simulink model "youBot_Arm_recovery"  (R2024a)
settings: Solver=ode15s  StartTime=0.0  StopTime=20  MaxStep=1e-2  RelTol=1e-3  AbsTol=1e-4
model workspace: external: MATLAB File youBot_DataFile.m (data not in the file)
undefined symbols (not defined in the file): Extr_Data_LinkHoles, Qt, s_curve_home2in, s_curve_in2out, s_curve_out2home, sigbuilder_block, smiData, X, Y, YBT_Par, Z
libraries: sm_lib x193, nesl_utility x130, fl_lib x53, simulink x13, Parts_Lib x10, MyMath_lib x8, Motor_Lib x5, Contact_Forces_Lib x4, ee_lib x2, sdl_lib x2
(part 8 of 8)

== system youBot_Arm_recovery/Arm/Environment/Conveyors/Belt In/Light Curtain/Geometry ==
  Beam 1 : sm_lib/Body Elements/Cylindrical Solid  CylinderRadius=beam_radius  CylinderRadiusUnits=m  CylinderLength=beam_length  CylinderLengthUnits=m  ExportEntireGeometry=off  InertiaType=CalculateFromGeometry  BasedOnType=Density  Density=1  DensityUnits=kg/m^3  Mass=1  MassUnits=kg  CenterOfMass=[0 0 0]  CenterOfMassUnits=m  MomentsOfInertia=[1 1 1]  MomentsOfInertiaUnits=kg*m^2  ProductsOfInertia=[1 1 1]  ProductsOfInertiaUnits=kg*m^2  GraphicType=FromGeometry  MarkerShape=Sphere  MarkerSize=10  GraphicVisPropType=SimpleVisualProperties  GraphicDiffuseColor=beam_color  GraphicOpacity=beam_opc  GraphicSpecularColor=[0.5 0.5 0.5 1.0]  GraphicAmbientColor=[0.15 0.15 0.15 1.0]  GraphicEmissiveColor=[0.0 0.0 0.0 1.0]  GraphicShininess=75  DoExposeReferenceFrame=on  SerializedFrames=<Frames/>
  Beam 2 : sm_lib/Body Elements/Cylindrical Solid  CylinderRadius=beam_radius  CylinderRadiusUnits=m  CylinderLength=beam_length  CylinderLengthUnits=m  ExportEntireGeometry=off  InertiaType=CalculateFromGeometry  BasedOnType=Density  Density=1  DensityUnits=kg/m^3  Mass=1  MassUnits=kg  CenterOfMass=[0 0 0]  CenterOfMassUnits=m  MomentsOfInertia=[1 1 1]  MomentsOfInertiaUnits=kg*m^2  ProductsOfInertia=[1 1 1]  ProductsOfInertiaUnits=kg*m^2  GraphicType=FromGeometry  MarkerShape=Sphere  MarkerSize=10  GraphicVisPropType=SimpleVisualProperties  GraphicDiffuseColor=beam_color  GraphicOpacity=beam_opc  GraphicSpecularColor=[0.5 0.5 0.5 1.0]  GraphicAmbientColor=[0.15 0.15 0.15 1.0]  GraphicEmissiveColor=[0.0 0.0 0.0 1.0]  GraphicShininess=75  DoExposeReferenceFrame=on  SerializedFrames=<Frames/>
  Beam 3 : sm_lib/Body Elements/Cylindrical Solid  CylinderRadius=beam_radius  CylinderRadiusUnits=m  CylinderLength=beam_length  CylinderLengthUnits=m  ExportEntireGeometry=off  InertiaType=CalculateFromGeometry  BasedOnType=Density  Density=1  DensityUnits=kg/m^3  Mass=1  MassUnits=kg  CenterOfMass=[0 0 0]  CenterOfMassUnits=m  MomentsOfInertia=[1 1 1]  MomentsOfInertiaUnits=kg*m^2  ProductsOfInertia=[1 1 1]  ProductsOfInertiaUnits=kg*m^2  GraphicType=FromGeometry  MarkerShape=Sphere  MarkerSize=10  GraphicVisPropType=SimpleVisualProperties  GraphicDiffuseColor=beam_color  GraphicOpacity=beam_opc  GraphicSpecularColor=[0.5 0.5 0.5 1.0]  GraphicAmbientColor=[0.15 0.15 0.15 1.0]  GraphicEmissiveColor=[0.0 0.0 0.0 1.0]  GraphicShininess=75  DoExposeReferenceFrame=on  SerializedFrames=<Frames/>
  Transform Beam 1 : sm_lib/Frames and Transforms/Rigid Transform  RotationMethod=None  FollAlignAxisA=+X  BaseAlignAxisA=+Y  FollAlignAxisB=+Y  BaseAlignAxisB=+Z  RotationStandardAxis=+Z  RotationAngle=0.0  RotationAngleUnits=deg  RotationArbitraryAxis=[0 0 1]  RotationSequenceAxes=FollowerAxes  RotationSequence=XYX  RotationSequenceAngles=[0 0 0]  RotationSequenceAnglesUnits=deg  RotationMatrix=[1 0 0; 0 1 0; 0 0 1]  Quaternion=[1 0 0 0]  TranslationMethod=StandardAxis  TranslationCartesianOffset=[0 0 0]  TranslationCartesianOffsetUnits=m  TranslationStandardAxis=-X  TranslationStandardOffset=YBT_Par.BeltIn.Sensor.Beam.offset  TranslationStandardOffsetUnits=m  TranslationROffset=0  TranslationROffsetUnits=m  TranslationThetaOffset=0  TranslationThetaOffsetUnits=deg  TranslationZOffset=0  TranslationZOffsetUnits=m
  Transform Beam 3 : sm_lib/Frames and Transforms/Rigid Transform  RotationMethod=None  FollAlignAxisA=+X  BaseAlignAxisA=+Y  FollAlignAxisB=+Y  BaseAlignAxisB=+Z  RotationStandardAxis=+Z  RotationAngle=0.0  RotationAngleUnits=deg  RotationArbitraryAxis=[0 0 1]  RotationSequenceAxes=FollowerAxes  RotationSequence=XYX  RotationSequenceAngles=[0 0 0]  RotationSequenceAnglesUnits=deg  RotationMatrix=[1 0 0; 0 1 0; 0 0 1]  Quaternion=[1 0 0 0]  TranslationMethod=StandardAxis  TranslationCartesianOffset=[0 0 0]  TranslationCartesianOffsetUnits=m  TranslationStandardAxis=-X  TranslationStandardOffset=YBT_Par.BeltIn.Sensor.Beam.offset  TranslationStandardOffsetUnits=m  TranslationROffset=0  TranslationROffsetUnits=m  TranslationThetaOffset=0  TranslationThetaOffsetUnits=deg  TranslationZOffset=0  TranslationZOffsetUnits=m
  Transform Orient z : sm_lib/Frames and Transforms/Rigid Transform  RotationMethod=AlignedAxes  FollAlignAxisA=+X  BaseAlignAxisA=+Z  FollAlignAxisB=+Z  BaseAlignAxisB=+Y  RotationStandardAxis=+X  RotationAngle=90  RotationAngleUnits=deg  RotationArbitraryAxis=[0 0 1]  RotationSequenceAxes=FollowerAxes  RotationSequence=XYX  RotationSequenceAngles=[0 0 0]  RotationSequenceAnglesUnits=deg  RotationMatrix=[1 0 0; 0 1 0; 0 0 1]  Quaternion=[1 0 0 0]  TranslationMethod=None  TranslationCartesianOffset=[0 0 0]  TranslationCartesianOffsetUnits=m  TranslationStandardAxis=+Z  TranslationStandardOffset=0  TranslationStandardOffsetUnits=m  TranslationROffset=0  TranslationROffsetUnits=m  TranslationThetaOffset=0  TranslationThetaOffsetUnits=deg  TranslationZOffset=0  TranslationZOffsetUnits=m
  R : PMIOPort  Side=Right
  connections:
  Beam 2/RConn1 -- Transform Orient z/RConn1 -- Transform Beam 1/RConn1 -- Transform Beam 3/LConn1
  Beam 1/RConn1 -- Transform Beam 1/LConn1
  Beam 3/RConn1 -- Transform Beam 3/RConn1
  Transform Orient z/LConn1 -- R/RConn1

== system youBot_Arm_recovery/Arm/Environment/Conveyors/Belt In/Light Curtain/Sensor ==
  note: Both sides
      | of sensor
  Abs : Abs  ZeroCross=off  SaturateOnIntegerOverflow=off
  Abs1 : Abs  ZeroCross=off  SaturateOnIntegerOverflow=off
  Abs2 : Abs  ZeroCross=off  SaturateOnIntegerOverflow=off
  Compare To Constant : simulink/Logic and Bit Operations/Compare To Constant  relop=<=  const=(YBT_Par.BeltIn.Sensor.Beam.length+YBT_Par.Cube.d)/2  OutDataTypeStr=boolean  ZeroCross=off
  Compare To Constant1 : simulink/Logic and Bit Operations/Compare To Constant  relop=<=  const=(YBT_Par.BeltIn.Sensor.Beam.radius*7+YBT_Par.Cube.d)/2  OutDataTypeStr=boolean  ZeroCross=off
  Compare To Constant2 : simulink/Logic and Bit Operations/Compare To Constant  relop=<=  const=(YBT_Par.BeltIn.Sensor.Beam.radius+YBT_Par.Cube.d)/2  OutDataTypeStr=boolean  ZeroCross=off
  Logical Operator : Logic  Operator=NAND  Inputs=3  AllPortsSameDT=off  OutDataTypeStr=boolean
  PS-Simulink Converter : nesl_utility/PS-Simulink Converter  PhysicalDomain=network_engine_domain  SubClassName=ps_output  LeftPortType=input  RightPortType=output  PseudoPeriodic=off  Frequencies=[]  VectorFormat=1-D array  Unit=1  AffineConversion=off
  PS-Simulink Converter1 : nesl_utility/PS-Simulink Converter  PhysicalDomain=network_engine_domain  SubClassName=ps_output  LeftPortType=input  RightPortType=output  PseudoPeriodic=off  Frequencies=[]  VectorFormat=1-D array  Unit=1  AffineConversion=off
  PS-Simulink Converter2 : nesl_utility/PS-Simulink Converter  PhysicalDomain=network_engine_domain  SubClassName=ps_output  LeftPortType=input  RightPortType=output  PseudoPeriodic=off  Frequencies=[]  VectorFormat=1-D array  Unit=1  AffineConversion=off
  Rigid Transform : sm_lib/Frames and Transforms/Rigid Transform  RotationMethod=AlignedAxes  FollAlignAxisA=+Y  BaseAlignAxisA=+Z  FollAlignAxisB=+X  BaseAlignAxisB=-X  RotationStandardAxis=+Z  RotationAngle=0.0  RotationAngleUnits=deg  RotationArbitraryAxis=[0 0 1]  RotationSequenceAxes=FollowerAxes  RotationSequence=XYX  RotationSequenceAngles=[0 0 0]  RotationSequenceAnglesUnits=deg  RotationMatrix=[1 0 0; 0 1 0; 0 0 1]  Quaternion=[1 0 0 0]  TranslationMethod=None  TranslationCartesianOffset=[0 0 0]  TranslationCartesianOffsetUnits=m  TranslationStandardAxis=+Z  TranslationStandardOffset=0  TranslationStandardOffsetUnits=m  TranslationROffset=0  TranslationROffsetUnits=m  TranslationThetaOffset=0  TranslationThetaOffsetUnits=deg  TranslationZOffset=0  TranslationZOffsetUnits=m
  Transform Sensor : sm_lib/Frames and Transforms/Transform Sensor  MeasurementFrame=Base  RotationSequence=XYX  SenseAngle=off  SenseAxis=off  SenseQ=off  SenseR=off  SenseRotationSequence=off  SenseOmegaX=off  SenseOmegaY=off  SenseOmegaZ=off  SenseOmega=off  SenseQDot=off  SenseRDot=off  SenseRotationSequenceDot=off  SenseAlphaX=off  SenseAlphaY=off  SenseAlphaZ=off  SenseAlpha=off  SenseQDDot=off  SenseRDDot=off  SenseX=on  SenseY=on  SenseZ=on  SenseXYZ=off  SenseRad=off  SenseAzim=off  SenseDist=off  SenseInc=off  SenseXDot=off  SenseYDot=off  SenseZDot=off  SenseXYZDot=off  SenseRadDot=off  SenseAzimDot=off  SenseDistDot=off  SenseIncDot=off  SenseXDDot=off  SenseYDDot=off  SenseZDDot=off  SenseXYZDDot=off  SenseRadDDot=off  SenseAzimDDot=off  SenseDistDDot=off  SenseIncDDot=off
  Unit Delay : UnitDelay  SampleTime=0.01  HasFrameUpgradeWarning=on
  F : PMIOPort  Side=Right
  B : PMIOPort  Port=2  Side=Left
  p : Outport  VectorParamsAs1DForOutWhenUnconnected=off
  wires:
  PS-Simulink Converter/1 -> Abs/1
  PS-Simulink Converter1/1 -> Abs1/1
  PS-Simulink Converter2/1 -> Abs2/1
  Abs1/1 -> Compare To Constant/1
  Abs2/1 -> Compare To Constant1/1
  Compare To Constant2/1 -> Logical Operator/1
  Compare To Constant/1 -> Logical Operator/2
  Compare To Constant1/1 -> Logical Operator/3
  Abs/1 -> Compare To Constant2/1
  Logical Operator/1 -> Unit Delay/1
  Unit Delay/1 -> p/1
  connections:
  PS-Simulink Converter2/LConn1 -- Transform Sensor/RConn4
  PS-Simulink Converter1/LConn1 -- Transform Sensor/RConn3
  PS-Simulink Converter/LConn1 -- Transform Sensor/RConn2
  F/RConn1 -- Transform Sensor/RConn1
  Rigid Transform/LConn1 -- B/RConn1
  Transform Sensor/LConn1 -- Rigid Transform/RConn1

== system youBot_Arm_recovery/Arm/Environment/Conveyors/Belt Out/Light Curtain/Geometry ==
  Beam 1 : sm_lib/Body Elements/Cylindrical Solid  CylinderRadius=beam_radius  CylinderRadiusUnits=m  CylinderLength=beam_length  CylinderLengthUnits=m  ExportEntireGeometry=off  InertiaType=CalculateFromGeometry  BasedOnType=Density  Density=1  DensityUnits=kg/m^3  Mass=1  MassUnits=kg  CenterOfMass=[0 0 0]  CenterOfMassUnits=m  MomentsOfInertia=[1 1 1]  MomentsOfInertiaUnits=kg*m^2  ProductsOfInertia=[1 1 1]  ProductsOfInertiaUnits=kg*m^2  GraphicType=FromGeometry  MarkerShape=Sphere  MarkerSize=10  GraphicVisPropType=SimpleVisualProperties  GraphicDiffuseColor=beam_color  GraphicOpacity=beam_opc  GraphicSpecularColor=[0.5 0.5 0.5 1.0]  GraphicAmbientColor=[0.15 0.15 0.15 1.0]  GraphicEmissiveColor=[0.0 0.0 0.0 1.0]  GraphicShininess=75  DoExposeReferenceFrame=on  SerializedFrames=<Frames/>
  Beam 2 : sm_lib/Body Elements/Cylindrical Solid  CylinderRadius=beam_radius  CylinderRadiusUnits=m  CylinderLength=beam_length  CylinderLengthUnits=m  ExportEntireGeometry=off  InertiaType=CalculateFromGeometry  BasedOnType=Density  Density=1  DensityUnits=kg/m^3  Mass=1  MassUnits=kg  CenterOfMass=[0 0 0]  CenterOfMassUnits=m  MomentsOfInertia=[1 1 1]  MomentsOfInertiaUnits=kg*m^2  ProductsOfInertia=[1 1 1]  ProductsOfInertiaUnits=kg*m^2  GraphicType=FromGeometry  MarkerShape=Sphere  MarkerSize=10  GraphicVisPropType=SimpleVisualProperties  GraphicDiffuseColor=beam_color  GraphicOpacity=beam_opc  GraphicSpecularColor=[0.5 0.5 0.5 1.0]  GraphicAmbientColor=[0.15 0.15 0.15 1.0]  GraphicEmissiveColor=[0.0 0.0 0.0 1.0]  GraphicShininess=75  DoExposeReferenceFrame=on  SerializedFrames=<Frames/>
  Beam 3 : sm_lib/Body Elements/Cylindrical Solid  CylinderRadius=beam_radius  CylinderRadiusUnits=m  CylinderLength=beam_length  CylinderLengthUnits=m  ExportEntireGeometry=off  InertiaType=CalculateFromGeometry  BasedOnType=Density  Density=1  DensityUnits=kg/m^3  Mass=1  MassUnits=kg  CenterOfMass=[0 0 0]  CenterOfMassUnits=m  MomentsOfInertia=[1 1 1]  MomentsOfInertiaUnits=kg*m^2  ProductsOfInertia=[1 1 1]  ProductsOfInertiaUnits=kg*m^2  GraphicType=FromGeometry  MarkerShape=Sphere  MarkerSize=10  GraphicVisPropType=SimpleVisualProperties  GraphicDiffuseColor=beam_color  GraphicOpacity=beam_opc  GraphicSpecularColor=[0.5 0.5 0.5 1.0]  GraphicAmbientColor=[0.15 0.15 0.15 1.0]  GraphicEmissiveColor=[0.0 0.0 0.0 1.0]  GraphicShininess=75  DoExposeReferenceFrame=on  SerializedFrames=<Frames/>
  Transform Beam 1 : sm_lib/Frames and Transforms/Rigid Transform  RotationMethod=None  FollAlignAxisA=+X  BaseAlignAxisA=+Y  FollAlignAxisB=+Y  BaseAlignAxisB=+Z  RotationStandardAxis=+Z  RotationAngle=0.0  RotationAngleUnits=deg  RotationArbitraryAxis=[0 0 1]  RotationSequenceAxes=FollowerAxes  RotationSequence=XYX  RotationSequenceAngles=[0 0 0]  RotationSequenceAnglesUnits=deg  RotationMatrix=[1 0 0; 0 1 0; 0 0 1]  Quaternion=[1 0 0 0]  TranslationMethod=StandardAxis  TranslationCartesianOffset=[0 0 0]  TranslationCartesianOffsetUnits=m  TranslationStandardAxis=-X  TranslationStandardOffset=YBT_Par.BeltIn.Sensor.Beam.offset  TranslationStandardOffsetUnits=m  TranslationROffset=0  TranslationROffsetUnits=m  TranslationThetaOffset=0  TranslationThetaOffsetUnits=deg  TranslationZOffset=0  TranslationZOffsetUnits=m
  Transform Beam 3 : sm_lib/Frames and Transforms/Rigid Transform  RotationMethod=None  FollAlignAxisA=+X  BaseAlignAxisA=+Y  FollAlignAxisB=+Y  BaseAlignAxisB=+Z  RotationStandardAxis=+Z  RotationAngle=0.0  RotationAngleUnits=deg  RotationArbitraryAxis=[0 0 1]  RotationSequenceAxes=FollowerAxes  RotationSequence=XYX  RotationSequenceAngles=[0 0 0]  RotationSequenceAnglesUnits=deg  RotationMatrix=[1 0 0; 0 1 0; 0 0 1]  Quaternion=[1 0 0 0]  TranslationMethod=StandardAxis  TranslationCartesianOffset=[0 0 0]  TranslationCartesianOffsetUnits=m  TranslationStandardAxis=-X  TranslationStandardOffset=YBT_Par.BeltIn.Sensor.Beam.offset  TranslationStandardOffsetUnits=m  TranslationROffset=0  TranslationROffsetUnits=m  TranslationThetaOffset=0  TranslationThetaOffsetUnits=deg  TranslationZOffset=0  TranslationZOffsetUnits=m
  Transform Orient z : sm_lib/Frames and Transforms/Rigid Transform  RotationMethod=AlignedAxes  FollAlignAxisA=+X  BaseAlignAxisA=+Z  FollAlignAxisB=+Z  BaseAlignAxisB=+Y  RotationStandardAxis=+X  RotationAngle=90  RotationAngleUnits=deg  RotationArbitraryAxis=[0 0 1]  RotationSequenceAxes=FollowerAxes  RotationSequence=XYX  RotationSequenceAngles=[0 0 0]  RotationSequenceAnglesUnits=deg  RotationMatrix=[1 0 0; 0 1 0; 0 0 1]  Quaternion=[1 0 0 0]  TranslationMethod=None  TranslationCartesianOffset=[0 0 0]  TranslationCartesianOffsetUnits=m  TranslationStandardAxis=+Z  TranslationStandardOffset=0  TranslationStandardOffsetUnits=m  TranslationROffset=0  TranslationROffsetUnits=m  TranslationThetaOffset=0  TranslationThetaOffsetUnits=deg  TranslationZOffset=0  TranslationZOffsetUnits=m
  R : PMIOPort  Side=Right
  connections:
  Transform Orient z/LConn1 -- R/RConn1
  Beam 3/RConn1 -- Transform Beam 3/RConn1
  Beam 1/RConn1 -- Transform Beam 1/LConn1
  Transform Orient z/RConn1 -- Beam 2/RConn1 -- Transform Beam 3/LConn1 -- Transform Beam 1/RConn1

== system youBot_Arm_recovery/Arm/Environment/Conveyors/Belt Out/Light Curtain/Sensor ==
  note: Both sides
      | of sensor
  Abs : Abs  ZeroCross=off  SaturateOnIntegerOverflow=off
  Abs1 : Abs  ZeroCross=off  SaturateOnIntegerOverflow=off
  Abs2 : Abs  ZeroCross=off  SaturateOnIntegerOverflow=off
  Compare To Constant : simulink/Logic and Bit Operations/Compare To Constant  relop=<=  const=(YBT_Par.BeltOut.Sensor.Beam.length+YBT_Par.Cube.d)/2  OutDataTypeStr=boolean  ZeroCross=off
  Compare To Constant1 : simulink/Logic and Bit Operations/Compare To Constant  relop=<=  const=(YBT_Par.BeltOut.Sensor.Beam.radius*7+YBT_Par.Cube.d)/2  OutDataTypeStr=boolean  ZeroCross=off
  Compare To Constant2 : simulink/Logic and Bit Operations/Compare To Constant  relop=<=  const=(YBT_Par.BeltOut.Sensor.Beam.radius+YBT_Par.Cube.d)/2  OutDataTypeStr=boolean  ZeroCross=off
  Logical Operator : Logic  Operator=NAND  Inputs=3  AllPortsSameDT=off  OutDataTypeStr=boolean
  PS-Simulink Converter : nesl_utility/PS-Simulink Converter  PhysicalDomain=network_engine_domain  SubClassName=ps_output  LeftPortType=input  RightPortType=output  PseudoPeriodic=off  Frequencies=[]  VectorFormat=1-D array  Unit=1  AffineConversion=off
  PS-Simulink Converter1 : nesl_utility/PS-Simulink Converter  PhysicalDomain=network_engine_domain  SubClassName=ps_output  LeftPortType=input  RightPortType=output  PseudoPeriodic=off  Frequencies=[]  VectorFormat=1-D array  Unit=1  AffineConversion=off
  PS-Simulink Converter2 : nesl_utility/PS-Simulink Converter  PhysicalDomain=network_engine_domain  SubClassName=ps_output  LeftPortType=input  RightPortType=output  PseudoPeriodic=off  Frequencies=[]  VectorFormat=1-D array  Unit=1  AffineConversion=off
  Rigid Transform : sm_lib/Frames and Transforms/Rigid Transform  RotationMethod=AlignedAxes  FollAlignAxisA=+Y  BaseAlignAxisA=+Z  FollAlignAxisB=+X  BaseAlignAxisB=-X  RotationStandardAxis=+Z  RotationAngle=0.0  RotationAngleUnits=deg  RotationArbitraryAxis=[0 0 1]  RotationSequenceAxes=FollowerAxes  RotationSequence=XYX  RotationSequenceAngles=[0 0 0]  RotationSequenceAnglesUnits=deg  RotationMatrix=[1 0 0; 0 1 0; 0 0 1]  Quaternion=[1 0 0 0]  TranslationMethod=None  TranslationCartesianOffset=[0 0 0]  TranslationCartesianOffsetUnits=m  TranslationStandardAxis=+Z  TranslationStandardOffset=0  TranslationStandardOffsetUnits=m  TranslationROffset=0  TranslationROffsetUnits=m  TranslationThetaOffset=0  TranslationThetaOffsetUnits=deg  TranslationZOffset=0  TranslationZOffsetUnits=m
  Transform Sensor : sm_lib/Frames and Transforms/Transform Sensor  MeasurementFrame=Base  RotationSequence=XYX  SenseAngle=off  SenseAxis=off  SenseQ=off  SenseR=off  SenseRotationSequence=off  SenseOmegaX=off  SenseOmegaY=off  SenseOmegaZ=off  SenseOmega=off  SenseQDot=off  SenseRDot=off  SenseRotationSequenceDot=off  SenseAlphaX=off  SenseAlphaY=off  SenseAlphaZ=off  SenseAlpha=off  SenseQDDot=off  SenseRDDot=off  SenseX=on  SenseY=on  SenseZ=on  SenseXYZ=off  SenseRad=off  SenseAzim=off  SenseDist=off  SenseInc=off  SenseXDot=off  SenseYDot=off  SenseZDot=off  SenseXYZDot=off  SenseRadDot=off  SenseAzimDot=off  SenseDistDot=off  SenseIncDot=off  SenseXDDot=off  SenseYDDot=off  SenseZDDot=off  SenseXYZDDot=off  SenseRadDDot=off  SenseAzimDDot=off  SenseDistDDot=off  SenseIncDDot=off
  Unit Delay : UnitDelay  SampleTime=0.01  HasFrameUpgradeWarning=on
  F : PMIOPort  Side=Right
  B : PMIOPort  Port=2  Side=Left
  p : Outport  VectorParamsAs1DForOutWhenUnconnected=off
  wires:
  Logical Operator/1 -> Unit Delay/1
  Abs/1 -> Compare To Constant2/1
  Compare To Constant1/1 -> Logical Operator/3
  Compare To Constant/1 -> Logical Operator/2
  Compare To Constant2/1 -> Logical Operator/1
  Abs2/1 -> Compare To Constant1/1
  Abs1/1 -> Compare To Constant/1
  PS-Simulink Converter2/1 -> Abs2/1
  PS-Simulink Converter1/1 -> Abs1/1
  PS-Simulink Converter/1 -> Abs/1
  Unit Delay/1 -> p/1
  connections:
  Transform Sensor/LConn1 -- Rigid Transform/RConn1
  Rigid Transform/LConn1 -- B/RConn1
  F/RConn1 -- Transform Sensor/RConn1
  PS-Simulink Converter/LConn1 -- Transform Sensor/RConn2
  PS-Simulink Converter1/LConn1 -- Transform Sensor/RConn3
  PS-Simulink Converter2/LConn1 -- Transform Sensor/RConn4

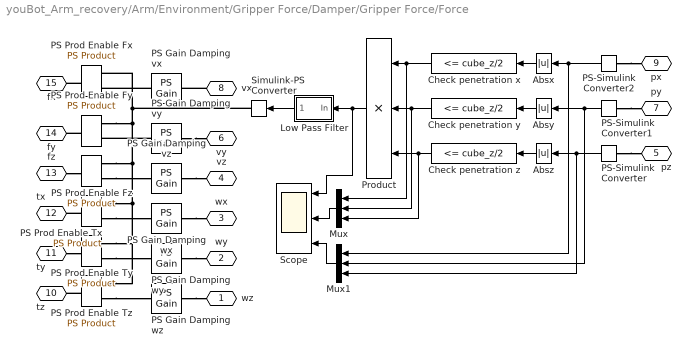
== system youBot_Arm_recovery/Arm/Environment/Gripper Force/Damper/Gripper Force/Force ==
  Absx : Abs  ZeroCross=off  SaturateOnIntegerOverflow=off
  Absy : Abs  ZeroCross=off  SaturateOnIntegerOverflow=off
  Absz : Abs  ZeroCross=off  SaturateOnIntegerOverflow=off
  Check penetration x : simulink/Logic and Bit Operations/Compare To Constant  relop=<=  const=cube_z/2  OutDataTypeStr=boolean  ZeroCross=off
  Check penetration y : simulink/Logic and Bit Operations/Compare To Constant  relop=<=  const=cube_z/2  OutDataTypeStr=boolean  ZeroCross=off
  Check penetration z : simulink/Logic and Bit Operations/Compare To Constant  relop=<=  const=cube_z/2  OutDataTypeStr=boolean  ZeroCross=off
  Low Pass Filter : Subsystem  mask(First-order lag supporting vector signals){b=lpfilt_const_force, x_initial=0}
      mask prompts: b "Filter time constant"; x_initial "Initial output"
      mask help: Models a lag of the form 1/(b*s+1) where s is the Laplace operator.
  Mux : Mux  Inputs=3
  Mux1 : Mux  Inputs=3
  PS Gain Damping vx : fl_lib/Physical Signals/Functions/PS Gain  gain=-contact_b N/(m/s)
  PS Gain Damping vy : fl_lib/Physical Signals/Functions/PS Gain  gain=-contact_b N/(m/s)
  PS Gain Damping vz : fl_lib/Physical Signals/Functions/PS Gain  gain=-contact_b N/(m/s)
  PS Gain Damping wx : fl_lib/Physical Signals/Functions/PS Gain  gain=-contact_b N*m/(rad/s)
  PS Gain Damping wy : fl_lib/Physical Signals/Functions/PS Gain  gain=-contact_b N*m/(rad/s)
  PS Gain Damping wz : fl_lib/Physical Signals/Functions/PS Gain  gain=-contact_b N*m/(rad/s)
  PS Prod Enable Fx : fl_lib/Physical Signals/Functions/PS Product
  PS Prod Enable Fy : fl_lib/Physical Signals/Functions/PS Product
  PS Prod Enable Fz : fl_lib/Physical Signals/Functions/PS Product
  PS Prod Enable Tx : fl_lib/Physical Signals/Functions/PS Product
  PS Prod Enable Ty : fl_lib/Physical Signals/Functions/PS Product
  PS Prod Enable Tz : fl_lib/Physical Signals/Functions/PS Product
  PS-Simulink Converter : nesl_utility/PS-Simulink Converter  PhysicalDomain=network_engine_domain  SubClassName=ps_output  LeftPortType=input  RightPortType=output  PseudoPeriodic=off  Frequencies=[]  VectorFormat=1-D array  Unit=1  AffineConversion=off
  PS-Simulink Converter1 : nesl_utility/PS-Simulink Converter  PhysicalDomain=network_engine_domain  SubClassName=ps_output  LeftPortType=input  RightPortType=output  PseudoPeriodic=off  Frequencies=[]  VectorFormat=1-D array  Unit=1  AffineConversion=off
  PS-Simulink Converter2 : nesl_utility/PS-Simulink Converter  PhysicalDomain=network_engine_domain  SubClassName=ps_output  LeftPortType=input  RightPortType=output  PseudoPeriodic=off  Frequencies=[]  VectorFormat=1-D array  Unit=1  AffineConversion=off
  Product : Product  Inputs=3  OutDataTypeStr=double
  Scope : Scope  NumInputPorts=3
  Simulink-PS Converter : nesl_utility/Simulink-PS Converter  PhysicalDomain=network_engine_domain  SubClassName=ps_input  LeftPortType=input  RightPortType=output  PseudoPeriodic=off  Frequencies=[]  NoiseDistribution=none  NoiseParameters=[]  Unit=1  AffineConversion=off  FilteringAndDerivatives=zero  SimscapeFilterOrder=1  InputFilterTimeConstant=0.005  UdotUserProvided=1
  wz : PMIOPort  Side=Left
  wy : PMIOPort  Port=2  Side=Left
  wx : PMIOPort  Port=3  Side=Left
  vz : PMIOPort  Port=4  Side=Left
  pz : PMIOPort  Port=5  Side=Left
  vy : PMIOPort  Port=6  Side=Left
  py : PMIOPort  Port=7  Side=Left
  vx : PMIOPort  Port=8  Side=Left
  px : PMIOPort  Port=9  Side=Left
  tz : PMIOPort  Port=10  Side=Right
  ty : PMIOPort  Port=11  Side=Right
  tx : PMIOPort  Port=12  Side=Right
  fz : PMIOPort  Port=13  Side=Right
  fy : PMIOPort  Port=14  Side=Right
  fx : PMIOPort  Port=15  Side=Right
  wires:
  PS-Simulink Converter1/1 -> Absy/1, Mux1/2
  PS-Simulink Converter2/1 -> Mux1/1, Absx/1
  Check penetration x/1 -> Mux/1, Product/1
  Check penetration y/1 -> Mux/2, Product/2
  Check penetration z/1 -> Mux/3, Product/3
  Mux/1 -> Scope/2
  Mux1/1 -> Scope/3
  PS-Simulink Converter/1 -> Mux1/3, Absz/1
  Absx/1 -> Check penetration x/1
  Absy/1 -> Check penetration y/1
  Absz/1 -> Check penetration z/1
  Product/1 -> Scope/1, Low Pass Filter/1(In)
  Low Pass Filter/1(Out) -> Simulink-PS Converter/1
  connections:
  vx/RConn1 -- PS Gain Damping vx/LConn1
  PS Gain Damping vx/RConn1 -- PS Prod Enable Fx/LConn2
  PS Gain Damping vy/RConn1 -- PS Prod Enable Fy/LConn2
  PS Gain Damping vy/LConn1 -- vy/RConn1
  PS Gain Damping vz/LConn1 -- vz/RConn1
  PS Prod Enable Fz/LConn2 -- PS Gain Damping vz/RConn1
  PS Prod Enable Tx/LConn2 -- PS Gain Damping wx/RConn1
  PS Gain Damping wx/LConn1 -- wx/RConn1
  PS Prod Enable Ty/LConn2 -- PS Gain Damping wy/RConn1
  PS Gain Damping wy/LConn1 -- wy/RConn1
  PS Prod Enable Tz/LConn2 -- PS Gain Damping wz/RConn1
  PS Gain Damping wz/LConn1 -- wz/RConn1
  PS-Simulink Converter/LConn1 -- pz/RConn1
  PS-Simulink Converter1/LConn1 -- py/RConn1
  PS-Simulink Converter2/LConn1 -- px/RConn1
  PS Prod Enable Tx/LConn1 -- PS Prod Enable Tz/LConn1 -- PS Prod Enable Ty/LConn1 -- PS Prod Enable Fz/LConn1 -- PS Prod Enable Fy/LConn1 -- PS Prod Enable Fx/LConn1 -- Simulink-PS Converter/RConn1
  PS Prod Enable Fx/RConn1 -- fx/RConn1
  PS Prod Enable Tz/RConn1 -- tz/RConn1
  ty/RConn1 -- PS Prod Enable Ty/RConn1
  PS Prod Enable Tx/RConn1 -- tx/RConn1
  fz/RConn1 -- PS Prod Enable Fz/RConn1
  PS Prod Enable Fy/RConn1 -- fy/RConn1

== system youBot_Arm_recovery/Arm/Environment/Gripper Force/Damper/Gripper Force/Relative vz ==
  Fingers : Subsystem  VariantControl=Fingers
  Housing : Subsystem  VariantControl=Housing
  vz fa : PMIOPort  Side=Left
  Box : PMIOPort  Port=2  Side=Left
  b : PMIOPort  Port=3  Side=Left
  E : PMIOPort  Port=4  Side=Left
  vz : PMIOPort  Port=5  Side=Right

== system youBot_Arm_recovery/Arm/Environment/Gripper Force/Damper/Gripper Force/Force/Low Pass Filter ==
  In : Inport
  Gain : Gain  Gain=1./b
  Integrator : Integrator  InitialCondition=x_initial.*b
  Sum : Sum  Inputs=|+-  InputSameDT=on  SaturateOnIntegerOverflow=on  OutDataTypeStr=Inherit: Same as first input
  Out : Outport  VectorParamsAs1DForOutWhenUnconnected=off
  wires:
  Sum/1 -> Integrator/1
  In/1 -> Sum/1
  Integrator/1 -> Gain/1
  Gain/1 -> Sum/2, Out/1

== system youBot_Arm_recovery/Arm/Environment/Gripper Force/Damper/Gripper Force/Relative vz/Fingers ==
  PS Gain2 : fl_lib/Physical Signals/Functions/PS Gain  gain=1
  PS Gain3 : fl_lib/Physical Signals/Functions/PS Gain  gain=1
  PS Subtract1 : fl_lib/Physical Signals/Functions/PS Subtract
  Transform Sensor : sm_lib/Frames and Transforms/Transform Sensor  MeasurementFrame=Base  RotationSequence=XYX  SenseAngle=off  SenseAxis=off  SenseQ=off  SenseR=off  SenseRotationSequence=off  SenseOmegaX=off  SenseOmegaY=off  SenseOmegaZ=off  SenseOmega=off  SenseQDot=off  SenseRDot=off  SenseRotationSequenceDot=off  SenseAlphaX=off  SenseAlphaY=off  SenseAlphaZ=off  SenseAlpha=off  SenseQDDot=off  SenseRDDot=off  SenseX=off  SenseY=off  SenseZ=off  SenseXYZ=off  SenseRad=off  SenseAzim=off  SenseDist=off  SenseInc=off  SenseXDot=off  SenseYDot=off  SenseZDot=on  SenseXYZDot=off  SenseRadDot=off  SenseAzimDot=off  SenseDistDot=off  SenseIncDot=off  SenseXDDot=off  SenseYDDot=off  SenseZDDot=off  SenseXYZDDot=off  SenseRadDDot=off  SenseAzimDDot=off  SenseDistDDot=off  SenseIncDDot=off
  vz fa : PMIOPort  Side=Left
  Box : PMIOPort  Port=2  Side=Left
  b : PMIOPort  Port=3  Side=Left
  E : PMIOPort  Port=4  Side=Left
  vz : PMIOPort  Port=5  Side=Right
  connections:
  PS Subtract1/LConn1 -- vz fa/RConn1
  PS Gain2/LConn1 -- Transform Sensor/RConn2
  Transform Sensor/LConn1 -- b/RConn1
  PS Gain3/LConn1 -- PS Subtract1/RConn1
  PS Subtract1/LConn2 -- PS Gain2/RConn1
  Transform Sensor/RConn1 -- Box/RConn1
  PS Gain3/RConn1 -- vz/RConn1

== system youBot_Arm_recovery/Arm/Environment/Gripper Force/Damper/Gripper Force/Relative vz/Housing ==
  PS Gain : fl_lib/Physical Signals/Functions/PS Gain  gain=1
  PS Terminator : fl_lib/Physical Signals/Sinks/PS Terminator
  Transform Sensor : sm_lib/Frames and Transforms/Transform Sensor  MeasurementFrame=Base  RotationSequence=XYX  SenseAngle=off  SenseAxis=off  SenseQ=off  SenseR=off  SenseRotationSequence=off  SenseOmegaX=off  SenseOmegaY=off  SenseOmegaZ=off  SenseOmega=off  SenseQDot=off  SenseRDot=off  SenseRotationSequenceDot=off  SenseAlphaX=off  SenseAlphaY=off  SenseAlphaZ=off  SenseAlpha=off  SenseQDDot=off  SenseRDDot=off  SenseX=off  SenseY=off  SenseZ=off  SenseXYZ=off  SenseRad=off  SenseAzim=off  SenseDist=off  SenseInc=off  SenseXDot=off  SenseYDot=off  SenseZDot=on  SenseXYZDot=off  SenseRadDot=off  SenseAzimDot=off  SenseDistDot=off  SenseIncDot=off  SenseXDDot=off  SenseYDDot=off  SenseZDDot=off  SenseXYZDDot=off  SenseRadDDot=off  SenseAzimDDot=off  SenseDistDDot=off  SenseIncDDot=off
  vz fa : PMIOPort  Side=Left
  Box : PMIOPort  Port=2  Side=Left
  b : PMIOPort  Port=3  Side=Left
  E : PMIOPort  Port=4  Side=Left
  vz : PMIOPort  Port=5  Side=Right
  connections:
  Transform Sensor/RConn1 -- Box/RConn1
  PS Gain/RConn1 -- vz/RConn1
  Transform Sensor/LConn1 -- E/RConn1
  PS Gain/LConn1 -- Transform Sensor/RConn2
  PS Terminator/LConn1 -- vz fa/RConn1

== stateflow chart youBot_Arm_recovery/Input/Control/Logic ==
  state BeltIn [parallel]
    settings: executionOrder=1
    state Empty
      entry:BeltIn_En = 0;
    state On
      entry:BeltIn_En=1;
    state BoxReady
      entry:Robot.GetBox
      BeltIn_En=0;
    state WaitClear
    (default) -> BeltIn.Empty
    (junction 133) -> BeltIn.Empty
    (junction 130) -> (junction 133)
    BeltIn.Empty -> BeltIn.On : [BeltIn_Box ==1]
    BeltIn.On -> BeltIn.BoxReady : [BeltIn_LC ==0]
    BeltIn.BoxReady -> BeltIn.WaitClear : [BeltIn_LC==1]
    BeltIn.WaitClear -> (junction 130) : after(delayBeltClear,sec)
  state Robot [parallel]
    settings: executionOrder=2
    state StartHome
      entry: Way=0;
    state GoBeltIn
      entry:Gripper.OpenGrip
      Way=1;
    state BeltIn
      entry:Gripper.GripBox
    state GoBeltOut
      entry:Way=2;
    state BeltOut
      entry:Gripper.DropBox
    state GoingHome
      entry:Way=3;
    state Home
      entry:Gripper.Close
    (default) -> StartHome
    StartHome -> GoBeltIn : GetBox
    (junction 138) -> GoBeltIn
    (junction 137) -> (junction 138)
    GoBeltIn -> Robot.BeltIn : after(delayGripBox,sec)
    Robot.BeltIn -> GoBeltOut : MoveBox
    GoBeltOut -> Robot.BeltOut : after(delayDropBox,sec)
    Robot.BeltOut -> GoingHome : GoHome
    GoingHome -> Home : after(delayClose,sec)
    Home -> (junction 137) : GetBox
  state Gripper [parallel]
    settings: executionOrder=3
    state Closed
      entry:Grip=0;
    state Open
      entry:Grip=1;
    state Tighten
      entry:Grip=2;
    state Grip
      entry:Robot.MoveBox
    state Release
      entry:Grip=1;
    (default) -> Closed
    Closed -> Open : OpenGrip
    Open -> Closed [order 2] : Close
    (junction 143) -> Open
    (junction 141) -> (junction 143)
    Open -> Tighten [order 1] : GripBox
    Tighten -> Grip : after(delayMoveBox,sec)
    Grip -> Release : DropBox
    Release -> (junction 141) : [after(delayShipBox,sec)]
        | {BeltOut.ShipBox}
  state BeltOut [parallel]
    settings: executionOrder=4
    state Empty
      entry:BeltOut_En = 0;
    state WaitRelease
    state On
      entry:BeltOut_En=1;
    state BoxReady
      entry:Robot.GoHome
      BeltOut_En=0;
    state WaitClear
    (default) -> BeltOut.Empty
    (junction 147) -> BeltOut.Empty
    (junction 146) -> (junction 147)
    BeltOut.Empty -> WaitRelease : [BeltOut_Box==1]
    WaitRelease -> BeltOut.On : ShipBox
    BeltOut.On -> BeltOut.BoxReady : [BeltOut_LC ==0]
    BeltOut.BoxReady -> BeltOut.WaitClear : [BeltOut_LC==1]
    BeltOut.WaitClear -> (junction 146) : after(delayBeltClear,sec)
  data: Way output; Grip output; BeltIn_Box input; BeltIn_LC input; BeltIn_En output; BeltOut_En output; BeltOut_Box input; BeltOut_LC input; delayClose parameter; delayDropBox parameter; delayBeltClear parameter; delayGripBox parameter; delayShipBox parameter; delayMoveBox parameter
  events: GetBox local FUNCTION_CALL_EVENT; MoveBox local FUNCTION_CALL_EVENT; GoHome local FUNCTION_CALL_EVENT; OpenGrip local FUNCTION_CALL_EVENT; GripBox local FUNCTION_CALL_EVENT; DropBox local FUNCTION_CALL_EVENT; Close local FUNCTION_CALL_EVENT; ShipBox local FUNCTION_CALL_EVENT
